simulink model "ThrottleArea"  (R2026a)
settings: Solver=VariableStepAuto
undefined symbols (not defined in the file): alpha0, alpha1
settings Model: Creator=flori  LastModifiedBy=flori

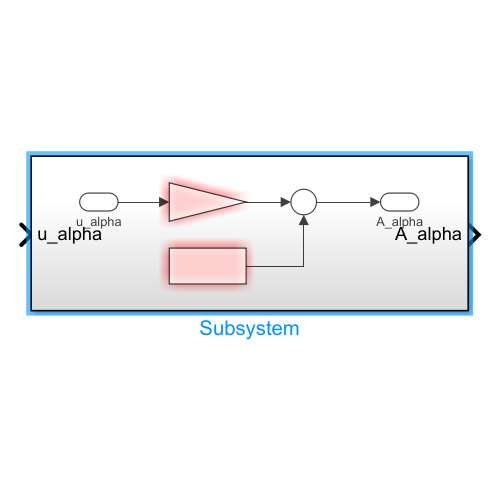
[thumbnail: Simulink's stored preview of the top-level diagram]
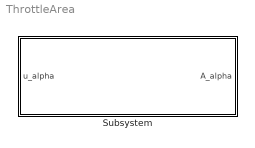
== system ThrottleArea ==
  Subsystem : Subsystem

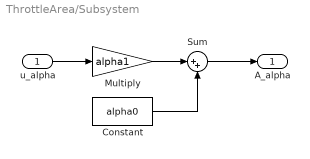
== system ThrottleArea/Subsystem ==
  u_alpha : Inport
  Constant : Constant  Value=alpha0
  Multiply : Gain  Gain=alpha1
  Sum : Sum  Inputs=|++
  A_alpha : Outport
  wires:
  Multiply/1 -> Sum/1
  Constant/1 -> Sum/2
  Sum/1 -> A_alpha/1
  u_alpha/1 -> Multiply/1
